simulink model "dynamic_of_reaction_wheel_backup"  (R2025a)
settings: Solver=VariableStepAuto  StartTime=0.0  StopTime=10  RelTol=1e-3
InitFcn:
  | run('D:\Work\Personal project\cubli\Matlab sim\Params.m');
values from neighbouring files (symbols this model uses):
  body_accel_gain = 1/IcO_bar    [Params.m]
  bw = 1.06e-5    (= 1.06e-05)    [Params.m]
  gravity_gain = mtot*g*d    [Params.m]
  tau_input = 0    [Params.m]
  wheel_accel_gain = 1/Iwg    (= 8000)    [Params.m]
settings Model: NumberOfSteps=5  Creator=Tran Anh Duy  LastModifiedBy=Tran Anh Duy

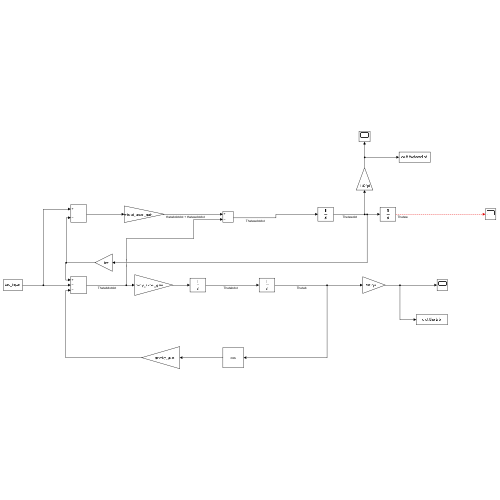
[thumbnail: Simulink's stored preview of the top-level diagram]
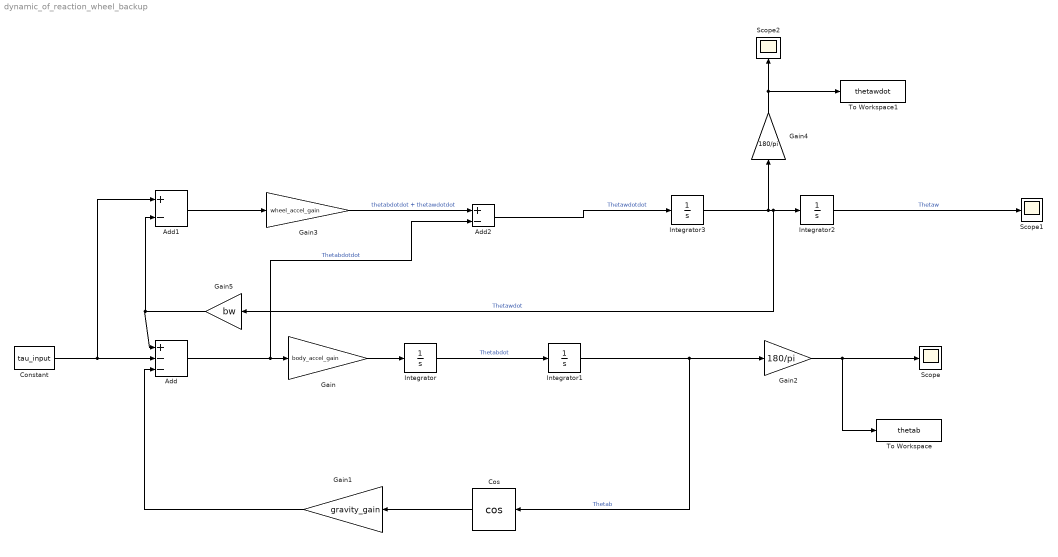
== system dynamic_of_reaction_wheel_backup ==
  Add : Sum  Inputs=+--
  Add1 : Sum  Inputs=+-
  Add2 : Sum  Inputs=+-
  Constant : Constant  Value=tau_input
  Cos : Trigonometry  Operator=cos
  Gain : Gain  Gain=body_accel_gain
  Gain1 : Gain  Gain=gravity_gain
  Gain2 : Gain  Gain=180/pi
  Gain3 : Gain  Gain=wheel_accel_gain
  Gain4 : Gain  Gain=180/pi
  Gain5 : Gain  Gain=bw
  Integrator : Integrator  InitialCondition=pi
  Integrator1 : Integrator
  Integrator2 : Integrator
  Integrator3 : Integrator
  Scope : Scope
      settings: ActiveDisplayYMinimum=-1.6385137887607009  ActiveDisplayYMaximum=4.8175477899719787
  Scope1 : Scope
      settings: ActiveDisplayYMinimum=-8882.6038169868243  ActiveDisplayYMaximum=79943.434352881435
  Scope2 : Scope
      settings: ActiveDisplayYMinimum=-716.22180359478023  ActiveDisplayYMaximum=6445.9962323530235  DataLoggingVariableName=ScopeData2
  To Workspace : ToWorkspace  VariableName=thetab  SampleTime=-1
  To Workspace1 : ToWorkspace  VariableName=thetawdot  SampleTime=-1
  wires:
  Add/1 -> Add2/2, Gain/1  "Thetabdotdot"
  Gain/1 -> Integrator/1
  Integrator/1 -> Integrator1/1  "Thetabdot"
  Integrator1/1 -> Cos/1, Gain2/1  "Thetab"
  Gain1/1 -> Add/3
  Constant/1 -> Add1/1, Add/2
  Integrator3/1 -> Gain4/1, Gain5/1, Integrator2/1  "Thetawdot"
  Integrator2/1 -> Scope1/1  "Thetaw"
  Add1/1 -> Gain3/1
  Cos/1 -> Gain1/1
  Gain2/1 -> To Workspace/1, Scope/1
  Gain5/1 -> Add1/2, Add/1
  Gain4/1 -> To Workspace1/1, Scope2/1
  Gain3/1 -> Add2/1  "thetabdotdot + thetawdotdot"
  Add2/1 -> Integrator3/1  "Thetawdotdot"
